simulink model "test_model"  (R2025a)
settings: Solver=VariableStepAuto  StartTime=0.0  StopTime=5  RelTol=1e-3
values from neighbouring files (symbols this model uses):
  K_dv = 15    [const.m]
  L_22 = 104    [const.m]
  m = 110    [const.m]
  U_max = 10    [const.m]
  V = 0.2    [const.m]
settings Model: Creator=Глеб  LastModifiedBy=Глеб

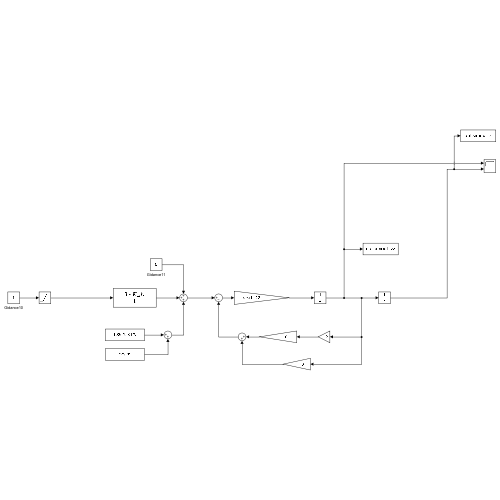
[thumbnail: Simulink's stored preview of the top-level diagram]
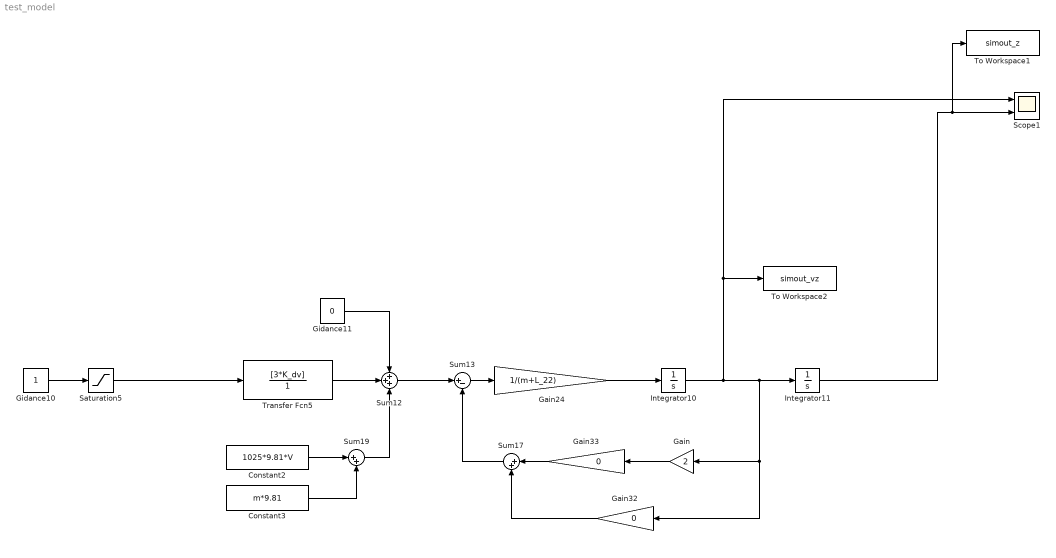
== system test_model ==
  Constant2 : Constant  Value=1025*9.81*V
  Constant3 : Constant  Value=m*9.81
  Gain : Gain  Gain=2
  Gain24 : Gain  Gain=1/(m+L_22)
  Gain32 : Gain  Gain=0
  Gain33 : Gain  Gain=0
  Gidance10 : Constant
  Gidance11 : Constant  Value=0
  Integrator10 : Integrator
  Integrator11 : Integrator
  Saturation5 : Saturate  UpperLimit=U_max  LowerLimit=-U_max
  Scope1 : Scope  NumInputPorts=2
      settings: ActiveDisplayYMinimum=-79.248200966048671  ActiveDisplayYMaximum=713.23380869443815
  Sum12 : Sum  Inputs=+++
  Sum13 : Sum  Inputs=|+-
  Sum17 : Sum  Inputs=|++
  Sum19 : Sum  Inputs=|++
  To Workspace1 : ToWorkspace  VariableName=simout_z  SaveFormat=Timeseries  SampleTime=-1
  To Workspace2 : ToWorkspace  VariableName=simout_vz  SaveFormat=Timeseries  SampleTime=-1
  Transfer Fcn5 : TransferFcn  Numerator=[3*K_dv]  Denominator=[0 1]
  wires:
  Gain24/1 -> Integrator10/1
  Gain33/1 -> Sum17/1
  Gain32/1 -> Sum17/2
  Gidance10/1 -> Saturation5/1
  Gidance11/1 -> Sum12/1
  Sum12/1 -> Sum13/1
  Integrator10/1 -> Scope1/1, To Workspace2/1, Gain/1, Gain32/1, Integrator11/1
  Constant2/1 -> Sum19/1
  Transfer Fcn5/1 -> Sum12/2
  Sum17/1 -> Sum13/2
  Integrator11/1 -> To Workspace1/1, Scope1/2
  Sum19/1 -> Sum12/3
  Constant3/1 -> Sum19/2
  Sum13/1 -> Gain24/1
  Saturation5/1 -> Transfer Fcn5/1
  Gain/1 -> Gain33/1
